simulink model "ex7"  (R2025b)
settings: Solver=FixedStepAuto  StartTime=0.0  StopTime=3  FixedStep=1e-5  RelTol=1e-3
values from neighbouring files (symbols this model uses):
  b = 0.001    [sim2.m]
  J = 0.05    [sim2.m]
  K = 1/sqrt(2)    [sim2.m]
  L_M = 0.20    (= 0.2)    [sim2.m]
  L_sig = 0.025    [sim2.m]
  np = p    (= 2)    [sim2.m]
  R_R = 0.45    [sim2.m]
  R_s = 1    [sim2.m]
  V_base = sqrt(2) * K * (V_n/sqrt(3))    [sim2.m]
  w_base = 2*pi*f_base    (= 314.159265359)    [sim2.m]
settings Model: Creator=dimit  LastModifiedBy=Dimitris

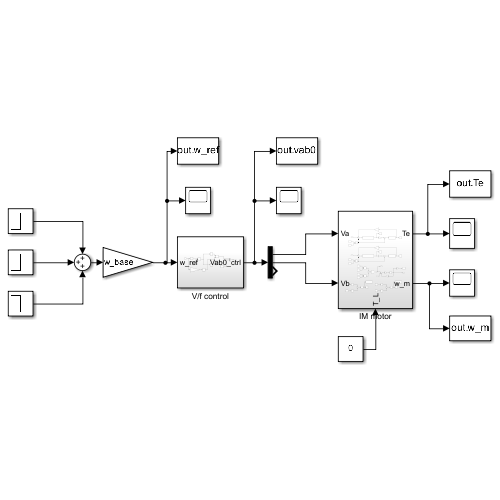
[thumbnail: Simulink's stored preview of the top-level diagram]
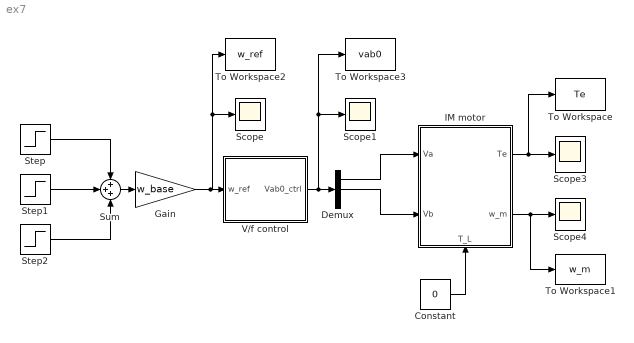
== system ex7 ==
  Constant : Constant  Value=0
  Demux : Demux  Outputs=3
  Gain : Gain  Gain=w_base
  IM motor : Subsystem
      settings: PortSchema="{\"entries\":[{\"content\":{\"sides\":[{\"content\":{\"connectorIds\":[\"In1\",\"In2\"]},\"type\":\"ConnectorPlacement.EquallySpacedRectSide\",\"uuid\":\"51ce8d8d-f70a-4d74-9403-4a2ac025a85e\"},{\"content\":{\"connectorIds\":[\"Out1\",\"Out2\"],\"side\":\"RIGHT\"},\"type\":\"ConnectorPlacement.EquallySpacedRectSide\",\"uuid\":\"f6ddc1dd-9c6b-4de5-b80a-02e3b764712c\"},{\"content\":{\"side\":\"TOP\"},\"type\":\"ConnectorPlacement.EquallySpacedRectSide\",\"uuid\":\"73a75396-5d1b-4b35-87ea-52b4d5235389\"},{\"content\":{\"connectorIds\":[\"In3\"],\"side\":\"BOTTOM\"},\"type\":\"ConnectorPlacement.EquallySpacedRectSide\",\"uuid\":\"d9589691-4817-4dea-b8b9-f2a79ff709eb\"}]},\"type\":\"ConnectorPlacement.EquallySpacedConnector\",\"uuid\":\"567b54d3-078a-47f2-aacd-44aae6ed51ca\"}],\"packageUris\":[\"http://schema.mathworks.com/mf0/Connector/R2020b\"],\"version\":\"1.0\"}"
  Scope{,1,3..4} (4 alike) : Scope
      Scope settings: ActiveDisplayYMinimum=-1  ActiveDisplayYMaximum=1
      Scope1 settings: ActiveDisplayYMinimum=-288.6751345948129  ActiveDisplayYMaximum=288.6751345948129
      Scope3 settings: ActiveDisplayYMinimum=-75.049842681006936  ActiveDisplayYMaximum=107.84432421320311  DataLoggingVariableName=ScopeData3
      Scope4 settings: ActiveDisplayYMinimum=-1  ActiveDisplayYMaximum=1  DataLoggingVariableName=ScopeData4
  Step : Step  Time=0.2  After=0.5  SampleTime=0
  Step1 : Step  Time=1.2  After=0.5  SampleTime=0
  Step2 : Step  Time=2  After=-1/3  SampleTime=0
  Sum : Sum  Inputs=+++
  To Workspace : ToWorkspace  VariableName=Te  SaveFormat=Timeseries  SampleTime=-1
  To Workspace1 : ToWorkspace  VariableName=w_m  SaveFormat=Timeseries  SampleTime=-1
  To Workspace2 : ToWorkspace  VariableName=w_ref  SaveFormat=Timeseries  SampleTime=-1
  To Workspace3 : ToWorkspace  VariableName=vab0  SaveFormat=Timeseries  SampleTime=-1
  V/f control : Subsystem
  wires:
  Demux/1 -> IM motor/1(Va)
  Demux/2 -> IM motor/2(Vb)
  IM motor/1(Te) -> To Workspace/1, Scope3/1
  V/f control/1(Vab0_ctrl) -> To Workspace3/1, Scope1/1, Demux/1
  Constant/1 -> IM motor/3(T_L)
  IM motor/2(w_m) -> To Workspace1/1, Scope4/1
  Step/1 -> Sum/1
  Step1/1 -> Sum/2
  Gain/1 -> To Workspace2/1, Scope/1, V/f control/1(w_ref)
  Sum/1 -> Gain/1
  Step2/1 -> Sum/3

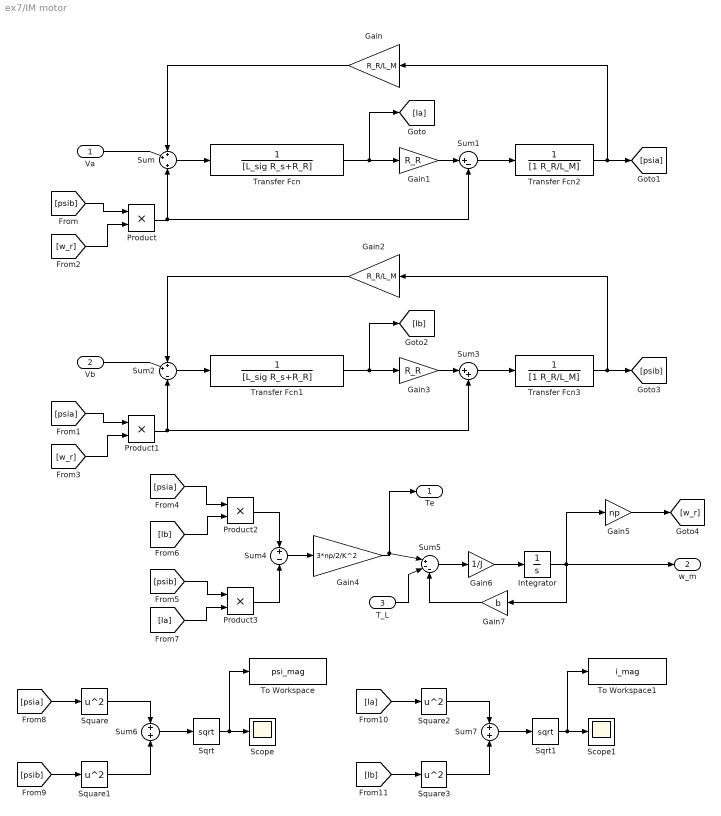
== system ex7/IM motor ==
  Va : Inport
  Vb : Inport  Port=2
  T_L : Inport  Port=3
  Gain : Gain  Gain=R_R/L_M
  Gain1 : Gain  Gain=R_R
  Gain2 : Gain  Gain=R_R/L_M
  Gain3 : Gain  Gain=R_R
  Gain4 : Gain  Gain=3*np/2/K^2
  Gain5 : Gain  Gain=np
  Gain6 : Gain  Gain=1/J
  Gain7 : Gain  Gain=b
  Integrator : Integrator
  Product{,1..3} (4 alike) : Product
  Scope : Scope
      settings: ActiveDisplayYMinimum=-1  ActiveDisplayYMaximum=1  DataLoggingVariableName=ScopeData5
  Scope1 : Scope
      settings: ActiveDisplayYMinimum=-8.05480318713023  ActiveDisplayYMaximum=72.493228684172081  DataLoggingVariableName=ScopeData6
  Sqrt : Sqrt
  Sqrt1 : Sqrt
  Square{,1..3} (4 alike) : Math  Operator=square
  Sum : Sum  Inputs=++|+
  Sum1 : Sum  Inputs=|+-
  Sum2 : Sum  Inputs=++|-
  Sum3 : Sum  Inputs=|++
  Sum4 : Sum  Inputs=+|-
  Sum5 : Sum  Inputs=|+--
  Sum6 : Sum
  Sum7 : Sum
  To Workspace : ToWorkspace  VariableName=psi_mag  SaveFormat=Timeseries  SampleTime=-1
  To Workspace1 : ToWorkspace  VariableName=i_mag  SaveFormat=Timeseries  SampleTime=-1
  Transfer Fcn : TransferFcn  Denominator=[L_sig R_s+R_R]
  Transfer Fcn1 : TransferFcn  Denominator=[L_sig R_s+R_R]
  Transfer Fcn2 : TransferFcn  Denominator=[1 R_R/L_M]
  Transfer Fcn3 : TransferFcn  Denominator=[1 R_R/L_M]
  Te : Outport
  w_m : Outport  Port=2
  wires:
  Sum/1 -> Transfer Fcn/1
  Transfer Fcn/1 -> [Ia], Gain1/1
  Transfer Fcn2/1 -> Gain/1, [psia]
  [psib] -> Product/1
  [w_r] -> Product/2
  Product/1 -> Sum1/2, Sum/3
  Gain1/1 -> Sum1/1
  Sum1/1 -> Transfer Fcn2/1
  Va/1 -> Sum/2
  Gain/1 -> Sum/1
  Vb/1 -> Sum2/2
  Transfer Fcn3/1 -> Gain2/1, [psib]
  Gain3/1 -> Sum3/1
  Product1/1 -> Sum3/2, Sum2/3
  Sum3/1 -> Transfer Fcn3/1
  [w_r] -> Product1/2
  Transfer Fcn1/1 -> [Ib], Gain3/1
  Sum2/1 -> Transfer Fcn1/1
  Gain2/1 -> Sum2/1
  [psia] -> Product1/1
  Gain4/1 -> Te/1, Sum5/1
  [psia] -> Product2/1
  [Ib] -> Product2/2
  Sum4/1 -> Gain4/1
  Product2/1 -> Sum4/1
  [psib] -> Product3/1
  [Ia] -> Product3/2
  Product3/1 -> Sum4/2
  T_L/1 -> Sum5/2
  Sum5/1 -> Gain6/1
  Integrator/1 -> Gain5/1, Gain7/1, w_m/1
  Gain5/1 -> [w_r]
  Square/1 -> Sum6/1
  Square1/1 -> Sum6/2
  Sum6/1 -> Sqrt/1
  Sqrt/1 -> To Workspace/1, Scope/1
  [psia] -> Square/1
  [psib] -> Square1/1
  [Ib] -> Square3/1
  Square3/1 -> Sum7/2
  Square2/1 -> Sum7/1
  Sum7/1 -> Sqrt1/1
  [Ia] -> Square2/1
  Sqrt1/1 -> To Workspace1/1, Scope1/1
  Gain6/1 -> Integrator/1
  Gain7/1 -> Sum5/3

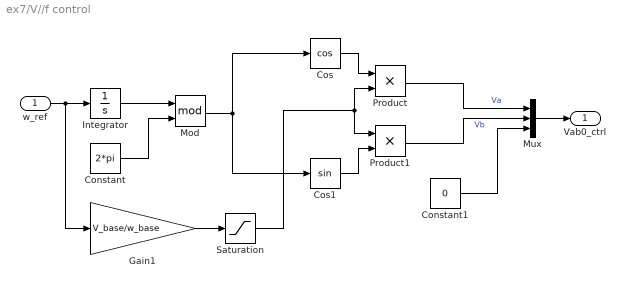
== system ex7/V//f control ==
  w_ref : Inport
  Constant : Constant  Value=2*pi
  Constant1 : Constant  Value=0
  Cos : Trigonometry  Operator=cos
  Cos1 : Trigonometry
  Gain1 : Gain  Gain=V_base/w_base
  Integrator : Integrator
  Mod : Math  Operator=mod
  Mux : Mux  Inputs=3
  Product : Product
  Product1 : Product
  Saturation : Saturate  UpperLimit=V_base  LowerLimit=-V_base
  Vab0_ctrl : Outport
  wires:
  Mux/1 -> Vab0_ctrl/1
  Constant/1 -> Mod/2
  Integrator/1 -> Mod/1
  Cos1/1 -> Product1/2
  Gain1/1 -> Saturation/1
  w_ref/1 -> Gain1/1, Integrator/1
  Mod/1 -> Cos1/1, Cos/1
  Cos/1 -> Product/1
  Saturation/1 -> Product1/1, Product/2
  Product/1 -> Mux/1  "Va"
  Product1/1 -> Mux/2  "Vb"
  Constant1/1 -> Mux/3
